simulink model "sldrtex_controller_4"  (R2015a)
settings: Solver=ode5  StartTime=0.0  StopTime=10.0  RelTol=1e-3
undefined symbols (not defined in the file): National_Instruments, PCI
libraries: sldrtlib x1
Description:
  | Real-Time Controller
  | 
  | This model shows how to build a simple closed-loop real-time controller using
  | Simulink Desktop Real-Time. The output of the controlled plant is connected
  | to the analog input of your data acquisition board. This signal is subtracted from
  | the set point value generated by the signal generator and processed by a PID
  | controller. The output of the controller drives the input of the plant using the analog
  | output of your data acquisition board.
  | 
  | This model is a simplified version of the controller used for the CE152 Magnetic
  | Levitation Model.
  | 
  | How to run this model in Normal Mode:
  | 
  | 1) Open the Analog Input and Analog Output blocks and select your data acquisition
  |    board. If there's no board installed, install it using the Install new board button.
  | 2) Double-click the orange button to switch to Normal Mode if needed.
  | 3) Start the real-time execution using Simulation->Run.
  | 
  | How to run this model in External Mode:
  | 
  | 1) Open the Analog Input and Analog Output blocks and select your data acquisition
  |    board. If there's no board installed, install it using the Install new board button.
  | 2) Double-click the orange button to switch to External Mode if needed.
  | 3) Start the real-time execution using Simulation->Run. The model will automatically
  |    build, connect to Simulink in External Mode and start.
  | 
  | Note:
  | To run this model, you must have a data acquisition board connected to your
  |    computer.
settings Model: CovSFcnEnable=off  ExtModeTrigDuration=10000  Creator=The MathWorks Inc.  LastModifiedBy=Aluno-05
settings DataIOCC: SignalLoggingName=logsOut
settings OptimizationCC: ExpressionDepthLimit=2147483647  InitFltsAndDblsToZero=on  EfficientMapNaN2IntZero=off
settings DebuggingCC: UnderspecifiedInitializationDetection=Classic  MergeDetectMultiDrivingBlocksExec=none  SignalResolutionControl=TryResolveAllWithWarning  FcnCallInpInsideContextMsg=UseLocalSettings  StateNameClashWarn=warning
settings HardwareCC: ProdBitPerLong=64  ProdBitPerPointer=64  ProdIntDivRoundTo=Zero  ProdEndianess=LittleEndian  ProdWordSize=64  ProdHWDeviceType=Intel->x86-64  TargetBitPerLong=64  TargetBitPerPointer=64  TargetIntDivRoundTo=Zero  TargetEndianess=LittleEndian  TargetWordSize=64  TargetHWDeviceType=Intel->x86-64
settings RTWCC: SystemTargetFile=rtwin.tlc  TemplateMakefile=rtwin.tmf  Description=Simulink Desktop Real-Time
settings RTWinTargetCC: TargetPreCompLibLocation=C:\Program Files\MATLAB\MATLAB Production Server\R2015a\toolbox\sldrt\lib\win64

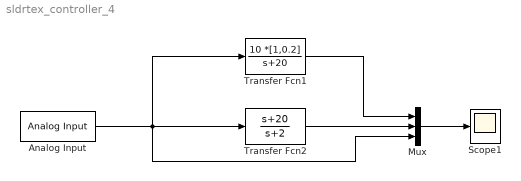
== system sldrtex_controller_4 ==
  Analog Input : sldrtlib/Analog Input  SampleTime=10e-3  MaxMissedTicks=20  ShowMissedTicks=off  YieldWhenWaiting=off  DrvName=National_Instruments/PCI-6221  DrvAddress=4294967295  DrvOptions=[0 0 0 0 0]  Channels=1  RangeMode=1  VoltRange=1  DataType=1
      settings: AttributesFormatString=National Instruments\nPCI-6221 [auto]
  Mux : Mux  Inputs=3
  Scope1 : Scope
      settings: TimeRange=10  YMin=-6  YMax=6  MaxDataPoints=10000  SampleInput=on  SampleTime=10e-3
  Transfer Fcn1 : TransferFcn  Numerator=10 *[1,0.2]  Denominator=[1, 20]
  Transfer Fcn2 : TransferFcn  Numerator=[1,20]  Denominator=[1, 2]
  wires:
  Analog Input/1 -> Transfer Fcn1/1, Transfer Fcn2/1, Mux/3
  Mux/1 -> Scope1/1
  Transfer Fcn1/1 -> Mux/1
  Transfer Fcn2/1 -> Mux/2
